simulink model "simulink4_inverted_pend_ss_model_wo_input"  (R2026b)
settings: Solver=ode113  StopTime=20.0  FixedStep=0.0001
values from neighbouring files (symbols this model uses):
  A = [0 0 1 0 ... (first row only)    [setup_inverted_pend_ss_model_wo_input.m]
  B = kt * B / Rm    [setup_inverted_pend_ss_model_wo_input.m]
  C = eye(4,4)    [setup_inverted_pend_ss_model_wo_input.m]
  D = zeros(4,1)    [setup_inverted_pend_ss_model_wo_input.m]
  K = place(A, B, p_desires)    [setup_inverted_pend_ss_model_wo_input.m]
  kr = 0    [setup_inverted_pend_ss_model_wo_input.m]
  x0 = [0.1; 0; 0; 0]    [setup_inverted_pend_ss_model_wo_input.m]
settings Model: Creator=leelou  LastModifiedBy=leelou

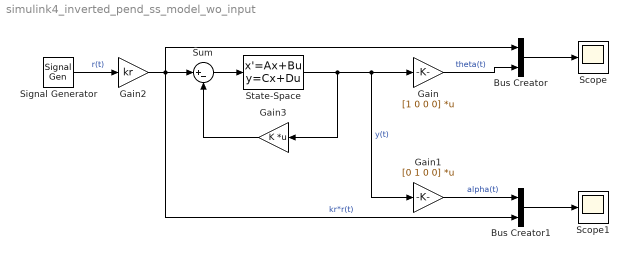
== system simulink4_inverted_pend_ss_model_wo_input ==
  Bus Creator : BusCreator  Inputs=2
  Bus Creator1 : BusCreator  Inputs=2
  Gain : Gain  Gain=[1 0 0 0]  Multiplication=Matrix(K*u) (u vector)
  Gain1 : Gain  Gain=[0 1 0 0]  Multiplication=Matrix(K*u) (u vector)
  Gain2 : Gain  Gain=kr
  Gain3 : Gain  Gain=K  Multiplication=Matrix(K*u) (u vector)
  Scope : Scope
      settings: ActiveDisplayYMinimum=-0.022377767087360743  ActiveDisplayYMaximum=0.12435623264667725
  Scope1 : Scope
      settings: ActiveDisplayYMinimum=-0.0046899944446366811  ActiveDisplayYMaximum=0.010873530027490034
  Signal Generator : SignalGenerator  WaveForm=square  Frequency=0.125
  State-Space : StateSpace  A=A  B=B  C=C  D=D  InitialCondition=x0
  Sum : Sum  Inputs=|+-
  wires:
  Bus Creator/1 -> Scope/1
  Signal Generator/1 -> Gain2/1  "r(t)"
  Bus Creator1/1 -> Scope1/1
  Gain1/1 -> Bus Creator1/1  "alpha(t)"
  Gain2/1 -> Bus Creator1/2, Bus Creator/1, Sum/1  "kr*r(t)"
  Sum/1 -> State-Space/1
  State-Space/1 -> Gain3/1, Gain1/1, Gain/1  "y(t)"
  Gain3/1 -> Sum/2
  Gain/1 -> Bus Creator/2  "theta(t)"
